simulink model "nms_sim_2D_cost"  (R2024b)
settings: Solver=ode15s  StartTime=0.0  StopTime=t_sim  MaxStep=dt_max  EnableMultiTasking=on
values from neighbouring files (symbols this model uses):
  a_BFSH = param_ctrl(35)*1    [setCtrlPar_optim_CPGreflex2001_2D.m]
  a_GAS = param_ctrl(37)*1    [setCtrlPar_optim_CPGreflex2001_2D.m]
  a_GLU = param_ctrl(31)*1    [setCtrlPar_optim_CPGreflex2001_2D.m]
  a_HAM = param_ctrl(33)*1    [setCtrlPar_optim_CPGreflex2001_2D.m]
  a_HFL = param_ctrl(32)*1    [setCtrlPar_optim_CPGreflex2001_2D.m]
  a_RF = param_ctrl(34)*1    [setCtrlPar_optim_CPGreflex2001_2D.m]
  a_SOL = param_ctrl(38)*1    [setCtrlPar_optim_CPGreflex2001_2D.m]
  a_TA = param_ctrl(39)*1    [setCtrlPar_optim_CPGreflex2001_2D.m]
  a_VAS = param_ctrl(36)*1    [setCtrlPar_optim_CPGreflex2001_2D.m]
  ai = param_ctrl(96)*2.0    [setCtrlPar_optim_CPGreflex2001_2D.m]
  b_BFSH = param_ctrl(52)*.51    [setCtrlPar_optim_CPGreflex2001_2D.m]
  b_BFSHGAS = param_ctrl(55)*.51    [setCtrlPar_optim_CPGreflex2001_2D.m]
  b_BFSHHAM = param_ctrl(54)*.51    [setCtrlPar_optim_CPGreflex2001_2D.m]
  b_BFSHVAS = param_ctrl(53)*.51    [setCtrlPar_optim_CPGreflex2001_2D.m]
  b_GAS = param_ctrl(59)*.51    [setCtrlPar_optim_CPGreflex2001_2D.m]
  b_GASBFSH = param_ctrl(60)*.51    [setCtrlPar_optim_CPGreflex2001_2D.m]
  b_GASSOL = param_ctrl(61)*.51    [setCtrlPar_optim_CPGreflex2001_2D.m]
  b_GLU = param_ctrl(40)*.51    [setCtrlPar_optim_CPGreflex2001_2D.m]
  b_GLUHAM = param_ctrl(42)*.51    [setCtrlPar_optim_CPGreflex2001_2D.m]
  b_GLUHFL = param_ctrl(41)*.51    [setCtrlPar_optim_CPGreflex2001_2D.m]
  b_HAM = param_ctrl(46)*.51    [setCtrlPar_optim_CPGreflex2001_2D.m]
  b_HAMBFSH = param_ctrl(48)*.51    [setCtrlPar_optim_CPGreflex2001_2D.m]
  b_HAMGLU = param_ctrl(47)*.51    [setCtrlPar_optim_CPGreflex2001_2D.m]
  b_HFL = param_ctrl(43)*.51    [setCtrlPar_optim_CPGreflex2001_2D.m]
  b_HFLGLU = param_ctrl(44)*.51    [setCtrlPar_optim_CPGreflex2001_2D.m]
  b_HFLRF = param_ctrl(45)*.51    [setCtrlPar_optim_CPGreflex2001_2D.m]
  b_RF = param_ctrl(49)*.51    [setCtrlPar_optim_CPGreflex2001_2D.m]
  b_RFHFL = param_ctrl(50)*.51    [setCtrlPar_optim_CPGreflex2001_2D.m]
  b_RFVAS = param_ctrl(51)*.51    [setCtrlPar_optim_CPGreflex2001_2D.m]
  b_SOL = param_ctrl(62)*.51    [setCtrlPar_optim_CPGreflex2001_2D.m]
  b_SOLGAS = param_ctrl(64)*.51    [setCtrlPar_optim_CPGreflex2001_2D.m]
  b_SOLTA = param_ctrl(63)*.51    [setCtrlPar_optim_CPGreflex2001_2D.m]
  b_TA = param_ctrl(65)*.51    [setCtrlPar_optim_CPGreflex2001_2D.m]
  b_TASOL = param_ctrl(66)*.51    [setCtrlPar_optim_CPGreflex2001_2D.m]
  b_VAS = param_ctrl(56)*.51    [setCtrlPar_optim_CPGreflex2001_2D.m]
  b_VASBFSH = param_ctrl(57)*.51    [setCtrlPar_optim_CPGreflex2001_2D.m]
  b_VASRF = param_ctrl(58)*.51    [setCtrlPar_optim_CPGreflex2001_2D.m]
  bias = param_ctrl(97)*2.5    [setCtrlPar_optim_CPGreflex2001_2D.m]
  c = 0.05    [nms_MS_2D_scaled.m]
  c_jointstop = 0.3 / (pi/180)    (= 17.1887338539)    [nms_MS_2D_scaled.m]
  D12_F = 0.16    *scaleL_JPhys    [nms_MechInit_2D_scaleSkel.m]
  D12_S = 0.2460	*sub_height    [nms_MechInit_2D_scaleSkel.m]
  D12_T = 0.2450  *sub_height    [nms_MechInit_2D_scaleSkel.m]
  D12y_F = 0.039  *sub_height    [nms_MechInit_2D_scaleSkel.m]
  D12z_HAT = 0.1    [nms_MS_2D_scaled.m]
  D13_F = 0.20    *scaleL_JPhys    [nms_MechInit_2D_scaleSkel.m]
  D1G_F = 0.14    *scaleL_JPhys    [nms_MechInit_2D_scaleSkel.m]
  D1G_HAT = 0.35  *scaleL_JPhys    [nms_MechInit_2D_scaleSkel.m]
  D1G_S = (0.3 - D12y_F/4)	*scaleL_JPhys    [nms_MechInit_2D_scaleSkel.m]
  D1G_T = (0.3 - D12y_F/4)	*scaleL_JPhys    [nms_MechInit_2D_scaleSkel.m]
  D1Gy_F = D12y_F*D1G_F/D12_F    (= 0.07)    [nms_MechInit_2D_scaleSkel.m]
  d_BFSH = param_ctrl(26)*1    [setCtrlPar_optim_CPGreflex2001_2D.m]
  d_GAS = param_ctrl(28)*1    [setCtrlPar_optim_CPGreflex2001_2D.m]
  d_GLU = param_ctrl(22)*1    [setCtrlPar_optim_CPGreflex2001_2D.m]
  d_HAM = param_ctrl(24)*1    [setCtrlPar_optim_CPGreflex2001_2D.m]
  d_HFL = param_ctrl(23)*1    [setCtrlPar_optim_CPGreflex2001_2D.m]
  d_RF = param_ctrl(25)*1    [setCtrlPar_optim_CPGreflex2001_2D.m]
  d_SOL = param_ctrl(29)*1    [setCtrlPar_optim_CPGreflex2001_2D.m]
  d_TA = param_ctrl(30)*1    [setCtrlPar_optim_CPGreflex2001_2D.m]
  d_VAS = param_ctrl(27)*1    [setCtrlPar_optim_CPGreflex2001_2D.m]
  DeltaThRef = 5e-3    (= 0.005)    [nms_MS_2D_scaled.m]
  dloptBFSH = 3.0    (= 3)    [setCtrlPar_optim_CPGreflex2001_2D.m]
  dloptGAS = 3.0    (= 3)    [setCtrlPar_optim_CPGreflex2001_2D.m]
  dloptGLU = 3.0    (= 3)    [setCtrlPar_optim_CPGreflex2001_2D.m]
  dloptHAM = 3.0    (= 3)    [setCtrlPar_optim_CPGreflex2001_2D.m]
  dloptHFL = 3.0    (= 3)    [setCtrlPar_optim_CPGreflex2001_2D.m]
  dloptRF = 3.0    (= 3)    [setCtrlPar_optim_CPGreflex2001_2D.m]
  dloptSOL = 3.0    (= 3)    [setCtrlPar_optim_CPGreflex2001_2D.m]
  dloptTA = 3.0    (= 3)    [setCtrlPar_optim_CPGreflex2001_2D.m]
  dloptVAS = 3.0    (= 3)    [setCtrlPar_optim_CPGreflex2001_2D.m]
  ec_BFSH = param_ctrl(80)*0.15    [setCtrlPar_optim_CPGreflex2001_2D.m]
  ec_GAS = param_ctrl(82)*0.15    [setCtrlPar_optim_CPGreflex2001_2D.m]
  ec_GLU = param_ctrl(76)*0.15    [setCtrlPar_optim_CPGreflex2001_2D.m]
  ec_HAM = param_ctrl(78)*0.15    [setCtrlPar_optim_CPGreflex2001_2D.m]
  ec_HFL = param_ctrl(77)*0.15    [setCtrlPar_optim_CPGreflex2001_2D.m]
  ec_RF = param_ctrl(79)*0.15    [setCtrlPar_optim_CPGreflex2001_2D.m]
  ec_TA = param_ctrl(84)*0.15    [setCtrlPar_optim_CPGreflex2001_2D.m]
  ec_VAS = param_ctrl(81)*0.15    [setCtrlPar_optim_CPGreflex2001_2D.m]
  eref = 0.04    [nms_MS_2D_scaled.m]
  eref_GAS = 0.1    [nms_MS_2D_scaled.m]
  eref_SOL = 0.1    [nms_MS_2D_scaled.m]
  es_BFSH = param_ctrl(89)*0.15    [setCtrlPar_optim_CPGreflex2001_2D.m]
  es_GAS = param_ctrl(91)*0.15    [setCtrlPar_optim_CPGreflex2001_2D.m]
  es_GLU = param_ctrl(85)*0.15    [setCtrlPar_optim_CPGreflex2001_2D.m]
  es_HAM = param_ctrl(87)*0.15    [setCtrlPar_optim_CPGreflex2001_2D.m]
  es_HFL = param_ctrl(86)*0.15    [setCtrlPar_optim_CPGreflex2001_2D.m]
  es_RF = param_ctrl(88)*0.15    [setCtrlPar_optim_CPGreflex2001_2D.m]
  es_TA = param_ctrl(93)*0.15    [setCtrlPar_optim_CPGreflex2001_2D.m]
  es_VAS = param_ctrl(90)*0.15    [setCtrlPar_optim_CPGreflex2001_2D.m]
  FmaxBFSH = 350    [nms_MS_2D_scaled.m]
  FmaxGAS = 2000    [nms_MS_2D_scaled.m]
  FmaxGLU = 4000    [nms_MS_2D_scaled.m]
  FmaxHAM = 2000    [nms_MS_2D_scaled.m]
  FmaxHFL = 2000    [nms_MS_2D_scaled.m]
  FmaxRF = 850    [nms_MS_2D_scaled.m]
  FmaxSOL = 4000    [nms_MS_2D_scaled.m]
  FmaxTA = 800    [nms_MS_2D_scaled.m]
  FmaxVAS = 5000    [nms_MS_2D_scaled.m]
  g = 9.81    [nms_MS_2D_scaled.m]
  gamma_4 = param_ctrl(11) * 1.7    [setCtrlPar_optim_CPGreflexsynergy2023_2D.m]
  h_BFSH = param_ctrl(71)*.1    [setCtrlPar_optim_CPGreflex2001_2D.m]
  h_GAS = param_ctrl(73)*.1    [setCtrlPar_optim_CPGreflex2001_2D.m]
  h_GLU = param_ctrl(67)*.1    [setCtrlPar_optim_CPGreflex2001_2D.m]
  h_HAM = param_ctrl(69)*.1    [setCtrlPar_optim_CPGreflex2001_2D.m]
  h_HFL = param_ctrl(68)*.1    [setCtrlPar_optim_CPGreflex2001_2D.m]
  h_RF = param_ctrl(70)*.1    [setCtrlPar_optim_CPGreflex2001_2D.m]
  h_SOL = param_ctrl(74)*.1    [setCtrlPar_optim_CPGreflex2001_2D.m]
  h_TA = param_ctrl(75)*.1    [setCtrlPar_optim_CPGreflex2001_2D.m]
  h_VAS = param_ctrl(72)*.1    [setCtrlPar_optim_CPGreflex2001_2D.m]
  HLCtrlPar = [theta_tgt l_clr alpha_tgt alpha_cd alpha_cv]    [setCtrlPar_optim_reflex2015_2D.m]
  In_F = 0.005    *scaleM*scaleL_JPhys^2    [nms_MechInit_2D_scaleSkel.m]
  In_HAT = 2.5    *scaleM*scaleL_JPhys^2    [nms_MechInit_2D_scaleSkel.m]
  In_S = 0.05     *scaleM*scaleL_JPhys^2    [nms_MechInit_2D_scaleSkel.m]
  In_T = 0.15     *scaleM*scaleL_JPhys^2    [nms_MechInit_2D_scaleSkel.m]
  init_exc = 0.01    [setInitPar_optim_2D.m]
  init_fm = 0.01    [setInitPar_optim_2D.m]
  init_lce = 1    [setInitPar_optim_2D.m]
  init_LCPG = param_ctrl(12) * 0.01    [setCtrlPar_optim_CPGreflexsynergy2023_2D.m]
  init_LStance = 1    [setInitPar_optim_2D.m]
  init_N1 = osc_signal1(phi_off_osc_ind)    [setCtrlPar_optim_CPGreflex2001_2D.m]
  ... (+441 more)
undefined symbols (not defined in the file or in its folder): cost_act_exponent, cost_v_tgt, flag_controller, Newton, nStep_obj, nStep_startKin, Raphson, sgn, SSW_kin, terrain_slope_angle, v_plateS1, X, Y, Z
libraries: nesl_utility x94, sm_lib x90, simulink x28, simulink_extras x12
(part 11 of 20)

== system nms_sim_2D_cost/Muscle Actuation/L BFSH ==
  note: BFSH Muscle-Tendon Dynamics
  note: Excitation Contraction Coupling
  A : Inport
  lmtc [m] : Inport  Port=2
  1 : Product  Inputs=**  InputSameDT=on  SaturateOnIntegerOverflow=on  OutDataTypeStr=Inherit: Same as first input
  1/lslack : Gain  Gain=1/lslackBFSH  SaturateOnIntegerOverflow=on  OutDataTypeStr=Inherit: Same as input  ParamDataTypeStr=Inherit: Same as input
  BE force-length relation : Subsystem
  CE force-length relation : Subsystem
  CE inverse force-velocity relation : Subsystem
  Constant : Constant  Value=lslackBFSH
  Fmax : Gain  Gain=FmaxBFSH  SaturateOnIntegerOverflow=on  OutDataTypeStr=Inherit: Same as input  ParamDataTypeStr=Inherit: Same as input
  Fmax1 : Gain  Gain=FmaxBFSH  SaturateOnIntegerOverflow=on  OutDataTypeStr=Inherit: Same as input  ParamDataTypeStr=Inherit: Same as input
  "Fpe = F^*pe * fv " : Product  InputSameDT=on  SaturateOnIntegerOverflow=on  OutDataTypeStr=Inherit: Same as first input
  Fv = Fse / (A*Fce) : Product  Inputs=*/  InputSameDT=on  SaturateOnIntegerOverflow=on  OutDataTypeStr=Inherit: Same as first input
  Integrator : Integrator  InitialConditionSource=external  LowerSaturationLimit=0.05
  PE force-length relation : Subsystem
  SE force-length relation : Subsystem
  Sum : Sum  Inputs=|+-  InputSameDT=on  SaturateOnIntegerOverflow=on  OutDataTypeStr=Inherit: Same as first input
  Sum1 : Sum  Inputs=|+-  InputSameDT=on  SaturateOnIntegerOverflow=on  OutDataTypeStr=Inherit: Same as first input
  Sum2 : Sum  Inputs=|-+  InputSameDT=on  SaturateOnIntegerOverflow=on  OutDataTypeStr=Inherit: Same as first input
  Sum3 : Sum  InputSameDT=on  SaturateOnIntegerOverflow=on  OutDataTypeStr=Inherit: Same as first input
  Sum4 : Sum  InputSameDT=on  SaturateOnIntegerOverflow=on  OutDataTypeStr=Inherit: Same as first input
  lce/lopt : Gain  Gain=1/loptBFSH  SaturateOnIntegerOverflow=on  OutDataTypeStr=Inherit: Same as input  ParamDataTypeStr=Inherit: Same as input
  vmax*lopt : Gain  Gain=vmaxBFSH*loptBFSH  SaturateOnIntegerOverflow=on  OutDataTypeStr=Inherit: Same as input  ParamDataTypeStr=Inherit: Same as input
  Fmtc : Outport  InitialOutput=0  VectorParamsAs1DForOutWhenUnconnected=off
  Lce : Outport  Port=2  InitialOutput=0  VectorParamsAs1DForOutWhenUnconnected=off
  Vce : Outport  Port=3  InitialOutput=0  VectorParamsAs1DForOutWhenUnconnected=off
  Fce : Outport  Port=4  InitialOutput=0  VectorParamsAs1DForOutWhenUnconnected=off
  lse [m] : Outport  Port=5  InitialOutput=0  VectorParamsAs1DForOutWhenUnconnected=off
  wires:
  Integrator/1 -> Sum/2, lce/lopt/1, Lce/1  "lce"
  lce/lopt/1 -> CE force-length relation/1(lce [lopt]), PE force-length relation/1(lce [lopt]), BE force-length relation/1(lce [lopt])
  Fv = Fse / (A*Fce)/1 -> "Fpe = F^*pe * fv "/1, CE inverse force-velocity relation/1(Fv[Fmax])  "fv"
  vmax*lopt/1 -> Integrator/1, Vce/1  "vce"
  lmtc [m]/1 -> Sum2/2, Sum/1  "lmtc"
  Fmax/1 -> Fmtc/1  "Fmtc"
  1/lslack/1 -> SE force-length relation/1(lse [lslack])
  SE force-length relation/1(fse [Fmax]) -> Fmax/1, Sum4/1
  Sum2/1 -> Integrator/2
  Constant/1 -> Sum2/1
  CE force-length relation/1(fce [Fmax]) -> 1/1
  PE force-length relation/1(fpe [Fmax]) -> "Fpe = F^*pe * fv "/2, Sum3/1
  1/1 -> Sum3/2
  BE force-length relation/1(fbe [Fmax]) -> Sum4/2
  Sum3/1 -> Fv = Fse / (A*Fce)/2
  CE inverse force-velocity relation/1(v[vmax]) -> vmax*lopt/1
  A/1 -> 1/2
  Sum4/1 -> Sum1/1, Fv = Fse / (A*Fce)/1  "Fse+Fbe"
  "Fpe = F^*pe * fv "/1 -> Sum1/2
  Sum1/1 -> Fmax1/1  "Fse+Fbe-Fpe"
  Fmax1/1 -> Fce/1
  Sum/1 -> lse [m]/1, 1/lslack/1  "lse"

== system nms_sim_2D_cost/Muscle Actuation/L BFSH Link ==
  note: BFSH Attachment
  phi23 [rad] : Inport
  Constant : Constant  Value=lslackBFSH+loptBFSH
  Constant1 : Constant  Value=rBFSH
  Constant2 : Constant  Value=phirefBFSH
  Gain4 : Gain  Gain=rhoBFSH
  Product : Product  RndMeth=Zero
  Sum2 : Sum  Inputs=|+-
  Sum5 : Sum  Inputs=|++
  lmtu [m] : Outport  VectorParamsAs1DForOutWhenUnconnected=off
  lever [m] : Outport  Port=2  VectorParamsAs1DForOutWhenUnconnected=off
  wires:
  Constant/1 -> Sum5/1
  Sum5/1 -> lmtu [m]/1
  Gain4/1 -> Sum5/2
  Product/1 -> Gain4/1
  phi23 [rad]/1 -> Sum2/1
  Constant2/1 -> Sum2/2
  Sum2/1 -> Product/1
  Constant1/1 -> Product/2, lever [m]/1

== system nms_sim_2D_cost/Muscle Actuation/L GAS ==
  note: SOLEUS Muscle-Tendon Dynamics
  note: Excitation Contraction Coupling
  A : Inport
  lmtc [m] : Inport  Port=2
  eref : Inport  Port=3
  1 : Product  Inputs=**  InputSameDT=on  SaturateOnIntegerOverflow=on  OutDataTypeStr=Inherit: Same as first input
  1/lslack : Gain  Gain=1/lslackGAS  SaturateOnIntegerOverflow=on  OutDataTypeStr=Inherit: Same as input  ParamDataTypeStr=Inherit: Same as input
  BE force-length relation : Subsystem
  CE force-length relation : Subsystem
  CE inverse force-velocity relation : Subsystem
  Constant : Constant  Value=lslackGAS
  Fmax : Gain  Gain=FmaxGAS  SaturateOnIntegerOverflow=on  OutDataTypeStr=Inherit: Same as input  ParamDataTypeStr=Inherit: Same as input
  Fmax1 : Gain  Gain=FmaxGAS  SaturateOnIntegerOverflow=on  OutDataTypeStr=Inherit: Same as input  ParamDataTypeStr=Inherit: Same as input
  "Fpe = F^*pe * fv " : Product  InputSameDT=on  SaturateOnIntegerOverflow=on  OutDataTypeStr=Inherit: Same as first input
  Fv = Fse / (A*Fce) : Product  Inputs=*/  InputSameDT=on  SaturateOnIntegerOverflow=on  OutDataTypeStr=Inherit: Same as first input
  Integrator : Integrator  InitialConditionSource=external  LowerSaturationLimit=0.05
  PE force-length relation : Subsystem
  SE force-length relation : Subsystem
  Sum : Sum  Inputs=|+-  InputSameDT=on  SaturateOnIntegerOverflow=on  OutDataTypeStr=Inherit: Same as first input
  Sum1 : Sum  Inputs=|+-  InputSameDT=on  SaturateOnIntegerOverflow=on  OutDataTypeStr=Inherit: Same as first input
  Sum2 : Sum  Inputs=|-+  InputSameDT=on  SaturateOnIntegerOverflow=on  OutDataTypeStr=Inherit: Same as first input
  Sum3 : Sum  InputSameDT=on  SaturateOnIntegerOverflow=on  OutDataTypeStr=Inherit: Same as first input
  Sum4 : Sum  InputSameDT=on  SaturateOnIntegerOverflow=on  OutDataTypeStr=Inherit: Same as first input
  lce/lopt : Gain  Gain=1/loptGAS  SaturateOnIntegerOverflow=on  OutDataTypeStr=Inherit: Same as input  ParamDataTypeStr=Inherit: Same as input
  vmax*lopt : Gain  Gain=vmaxGAS*loptGAS  SaturateOnIntegerOverflow=on  OutDataTypeStr=Inherit: Same as input  ParamDataTypeStr=Inherit: Same as input
  Fmtc : Outport  InitialOutput=0  VectorParamsAs1DForOutWhenUnconnected=off
  Lce : Outport  Port=2  InitialOutput=0  VectorParamsAs1DForOutWhenUnconnected=off
  Vce : Outport  Port=3  InitialOutput=0  VectorParamsAs1DForOutWhenUnconnected=off
  Fce : Outport  Port=4  InitialOutput=0  VectorParamsAs1DForOutWhenUnconnected=off
  lse [m] : Outport  Port=5  InitialOutput=0  VectorParamsAs1DForOutWhenUnconnected=off
  wires:
  Integrator/1 -> Sum/2, lce/lopt/1, Lce/1  "lce"
  lce/lopt/1 -> CE force-length relation/1(lce [lopt]), PE force-length relation/1(lce [lopt]), BE force-length relation/1(lce [lopt])
  Fv = Fse / (A*Fce)/1 -> "Fpe = F^*pe * fv "/1, CE inverse force-velocity relation/1(Fv[Fmax])  "fv"
  vmax*lopt/1 -> Integrator/1, Vce/1  "vce"
  lmtc [m]/1 -> Sum2/2, Sum/1  "lmtc"
  Fmax/1 -> Fmtc/1  "Fmtc"
  1/lslack/1 -> SE force-length relation/1(lse [lslack])
  SE force-length relation/1(fse [Fmax]) -> Fmax/1, Sum4/1
  Sum2/1 -> Integrator/2
  Constant/1 -> Sum2/1
  CE force-length relation/1(fce [Fmax]) -> 1/1
  PE force-length relation/1(fpe [Fmax]) -> "Fpe = F^*pe * fv "/2, Sum3/1
  1/1 -> Sum3/2
  BE force-length relation/1(fbe [Fmax]) -> Sum4/2
  Sum3/1 -> Fv = Fse / (A*Fce)/2
  CE inverse force-velocity relation/1(v[vmax]) -> vmax*lopt/1
  A/1 -> 1/2
  Sum4/1 -> Sum1/1, Fv = Fse / (A*Fce)/1  "Fse+Fbe"
  "Fpe = F^*pe * fv "/1 -> Sum1/2
  Sum1/1 -> Fmax1/1  "Fse+Fbe-Fpe"
  Fmax1/1 -> Fce/1
  Sum/1 -> lse [m]/1, 1/lslack/1  "lse"
  eref/1 -> SE force-length relation/2(eref)

== system nms_sim_2D_cost/Muscle Actuation/L GAS Link ==
  note: GAS Attachment
  phi23 [rad] : Inport
  phi12 [rad] : Inport  Port=2
  Constant1 : Constant  Value=phimaxGASk
  Constant2 : Constant  Value=phirefGASk
  Constant3 : Constant  Value=phimaxGASa
  Constant4 : Constant  Value=lslackGAS+loptGAS
  Constant5 : Constant  Value=phirefGASa
  Demux : Demux  Outputs=2
  Demux1 : Demux  Outputs=2
  Gain1 : Gain  Gain=rGASkmax
  Gain2 : Gain  Gain=rGASamax
  Gain3 : Gain  Gain=phiScaleGASa
  Gain5 : Gain  Gain=phiScaleGASk
  Gain6 : Gain  Gain=phiScaleGASk
  Gain7 : Gain  Gain=rhoGASk/phiScaleGASk
  Gain8 : Gain  Gain=phiScaleGASa
  Gain9 : Gain  Gain=rhoGASa/phiScaleGASa
  Mux : Mux  Inputs=2
  Mux1 : Mux  Inputs=2
  Sum1 : Sum  Inputs=-+
  Sum2 : Sum  Inputs=|+-
  Sum3 : Sum  Inputs=-+|
  Sum4 : Sum  Inputs=-+
  Sum5 : Sum  Inputs=++-
  Sum6 : Sum  Inputs=|+-
  Sum7 : Sum  Inputs=-+|
  length change term : Trigonometry
  length change term1 : Trigonometry
  offset correction term : Trigonometry
  offset correction term1 : Trigonometry
  variable lever term : Trigonometry  Operator=cos
  variable lever term1 : Trigonometry  Operator=cos
  lmtu [m] : Outport  VectorParamsAs1DForOutWhenUnconnected=off
  lever23 [m] : Outport  Port=2  VectorParamsAs1DForOutWhenUnconnected=off
  lever12 [m] : Outport  Port=3  VectorParamsAs1DForOutWhenUnconnected=off
  wires:
  Sum5/1 -> lmtu [m]/1
  Demux1/2 -> lever12 [m]/1
  Constant4/1 -> Sum5/2
  Demux1/1 -> Gain9/1
  Gain9/1 -> Sum5/3
  Demux/2 -> lever23 [m]/1
  Demux/1 -> Gain7/1
  Gain7/1 -> Sum5/1
  phi23 [rad]/1 -> Sum3/2
  Sum3/1 -> Gain5/1
  Constant1/1 -> Sum3/1, Sum2/2
  Sum2/1 -> Gain6/1
  Constant2/1 -> Sum2/1
  length change term/1 -> Sum1/2
  offset correction term/1 -> Sum1/1
  Sum1/1 -> Mux/1
  variable lever term/1 -> Mux/2
  Mux/1 -> Gain1/1
  Gain1/1 -> Demux/1
  Gain5/1 -> variable lever term/1, length change term/1
  Gain6/1 -> offset correction term/1
  phi12 [rad]/1 -> Sum7/2
  Sum7/1 -> Gain3/1
  Constant3/1 -> Sum7/1, Sum6/2
  Sum6/1 -> Gain8/1
  Constant5/1 -> Sum6/1
  length change term1/1 -> Sum4/2
  offset correction term1/1 -> Sum4/1
  Sum4/1 -> Mux1/1
  variable lever term1/1 -> Mux1/2
  Mux1/1 -> Gain2/1
  Gain2/1 -> Demux1/1
  Gain3/1 -> variable lever term1/1, length change term1/1
  Gain8/1 -> offset correction term1/1

== system nms_sim_2D_cost/Muscle Actuation/L Hip Joint Limits ==
  note: Hip Joint Limits
  phi [rad] : Inport
  dphi [rad/s] : Inport  Port=2
  Gain1 : Gain  Gain=c_jointstop
  Gain2 : Gain  Gain=-1
  Gain3 : Gain  Gain=c_jointstop
  Gain4 : Gain  Gain=1/w_max_jointstop
  Limit Ankle Range : simulink/Logic and Bit Operations/Interval Test  Commented=on  IntervalClosedRight=on  uplimit=phi12_UpLimit + 40*pi/180  IntervalClosedLeft=on  lowlimit=phi12_LowLimit - 40*pi/180  OutDataTypeStr=boolean
  Logical Operator3 : Logic  Commented=on  Operator=NOT  AllPortsSameDT=off  OutDataTypeStr=boolean
  Mux1 : Mux  Inputs=2
  Mux3 : Mux  Inputs=2
  Overextension Torque : Fcn  Expr="- u(1)  *  (1-u(2)) * (u(2)<1) * (u(1)>0)"
  Overflexion Torque : Fcn  Expr="- u(1)  *  (1-u(2)) * (u(2)<1) * (u(1)<0)"
  Stop Simulation1 : Stop  Commented=on
  Sum : Sum  Inputs=|+-
  Sum1 : Sum  Inputs=|+-
  Sum2 : Sum
  overextension angle : Constant  Value=phi34_UpLimit
  overflexion angle : Constant  Value=phi34_LowLimit
  M_stop [Nm] : Outport  VectorParamsAs1DForOutWhenUnconnected=off
  wires:
  Mux3/1 -> Overextension Torque/1
  Gain3/1 -> Mux3/1
  dphi [rad/s]/1 -> Gain4/1
  overextension angle/1 -> Sum/2
  phi [rad]/1 -> Sum/1, Sum1/1, Limit Ankle Range/1
  Sum/1 -> Gain3/1
  Gain4/1 -> Gain2/1, Mux1/2
  Gain1/1 -> Mux1/1
  Sum1/1 -> Gain1/1
  overflexion angle/1 -> Sum1/2
  Mux1/1 -> Overflexion Torque/1
  Sum2/1 -> M_stop [Nm]/1
  Gain2/1 -> Mux3/2
  Overflexion Torque/1 -> Sum2/2
  Overextension Torque/1 -> Sum2/1
  Limit Ankle Range/1 -> Logical Operator3/1
  Logical Operator3/1 -> Stop Simulation1/1

== system nms_sim_2D_cost/Muscle Actuation/L Knee Joint Limits ==
  note: Knee Joint Limits
  phi [rad] : Inport
  dphi [rad/s] : Inport  Port=2
  Gain1 : Gain  Gain=c_jointstop
  Gain2 : Gain  Gain=-1
  Gain3 : Gain  Gain=c_jointstop
  Gain4 : Gain  Gain=1/w_max_jointstop
  Limit Ankle Range : simulink/Logic and Bit Operations/Interval Test  Commented=on  IntervalClosedRight=on  uplimit=phi12_UpLimit + 40*pi/180  IntervalClosedLeft=on  lowlimit=phi12_LowLimit - 40*pi/180  OutDataTypeStr=boolean
  Logical Operator3 : Logic  Commented=on  Operator=NOT  AllPortsSameDT=off  OutDataTypeStr=boolean
  Mux1 : Mux  Inputs=2
  Mux3 : Mux  Inputs=2
  Overextension Torque : Fcn  Expr="- u(1)  *  (1-u(2)) * (u(2)<1) * (u(1)>0)"
  Overflexion Torque : Fcn  Expr="- u(1)  *  (1-u(2)) * (u(2)<1) * (u(1)<0)"
  Stop Simulation1 : Stop  Commented=on
  Sum : Sum  Inputs=|+-
  Sum1 : Sum  Inputs=|+-
  Sum2 : Sum
  overextension angle : Constant  Value=phi23_UpLimit
  overflexion angle : Constant  Value=phi23_LowLimit
  M_stop [Nm] : Outport  VectorParamsAs1DForOutWhenUnconnected=off
  wires:
  Mux3/1 -> Overextension Torque/1
  Gain3/1 -> Mux3/1
  dphi [rad/s]/1 -> Gain4/1
  overextension angle/1 -> Sum/2
  phi [rad]/1 -> Sum/1, Sum1/1, Limit Ankle Range/1
  Sum/1 -> Gain3/1
  Gain4/1 -> Gain2/1, Mux1/2
  Gain1/1 -> Mux1/1
  Sum1/1 -> Gain1/1
  overflexion angle/1 -> Sum1/2
  Mux1/1 -> Overflexion Torque/1
  Sum2/1 -> M_stop [Nm]/1
  Gain2/1 -> Mux3/2
  Overflexion Torque/1 -> Sum2/2
  Overextension Torque/1 -> Sum2/1
  Limit Ankle Range/1 -> Logical Operator3/1
  Logical Operator3/1 -> Stop Simulation1/1

== system nms_sim_2D_cost/Muscle Actuation/L SOL ==
  note: SOLEUS Muscle-Tendon Dynamics
  note: Excitation Contraction Coupling
  A : Inport
  lmtc [m] : Inport  Port=2
  eref : Inport  Port=3
  1 : Product  Inputs=**  InputSameDT=on  SaturateOnIntegerOverflow=on  OutDataTypeStr=Inherit: Same as first input
  1/lslack : Gain  Gain=1/lslackSOL  SaturateOnIntegerOverflow=on  OutDataTypeStr=Inherit: Same as input  ParamDataTypeStr=Inherit: Same as input
  BE force-length relation : Subsystem
  CE force-length relation : Subsystem
  CE inverse force-velocity relation : Subsystem
  Constant : Constant  Value=lslackSOL
  Fmax : Gain  Gain=FmaxSOL  SaturateOnIntegerOverflow=on  OutDataTypeStr=Inherit: Same as input  ParamDataTypeStr=Inherit: Same as input
  Fmax1 : Gain  Gain=FmaxSOL  SaturateOnIntegerOverflow=on  OutDataTypeStr=Inherit: Same as input  ParamDataTypeStr=Inherit: Same as input
  "Fpe = F^*pe * fv " : Product  InputSameDT=on  SaturateOnIntegerOverflow=on  OutDataTypeStr=Inherit: Same as first input
  Fv = Fse / (A*Fce) : Product  Inputs=*/  InputSameDT=on  SaturateOnIntegerOverflow=on  OutDataTypeStr=Inherit: Same as first input
  Integrator : Integrator  InitialConditionSource=external  LowerSaturationLimit=0.05
  PE force-length relation : Subsystem
  SE force-length relation : Subsystem
  Sum : Sum  Inputs=|+-  InputSameDT=on  SaturateOnIntegerOverflow=on  OutDataTypeStr=Inherit: Same as first input
  Sum1 : Sum  Inputs=|+-  InputSameDT=on  SaturateOnIntegerOverflow=on  OutDataTypeStr=Inherit: Same as first input
  Sum2 : Sum  Inputs=|-+  InputSameDT=on  SaturateOnIntegerOverflow=on  OutDataTypeStr=Inherit: Same as first input
  Sum3 : Sum  InputSameDT=on  SaturateOnIntegerOverflow=on  OutDataTypeStr=Inherit: Same as first input
  Sum4 : Sum  InputSameDT=on  SaturateOnIntegerOverflow=on  OutDataTypeStr=Inherit: Same as first input
  lce/lopt : Gain  Gain=1/loptSOL  SaturateOnIntegerOverflow=on  OutDataTypeStr=Inherit: Same as input  ParamDataTypeStr=Inherit: Same as input
  vmax*lopt : Gain  Gain=vmaxSOL*loptSOL  SaturateOnIntegerOverflow=on  OutDataTypeStr=Inherit: Same as input  ParamDataTypeStr=Inherit: Same as input
  Fmtc : Outport  InitialOutput=0  VectorParamsAs1DForOutWhenUnconnected=off
  Lce : Outport  Port=2  InitialOutput=0  VectorParamsAs1DForOutWhenUnconnected=off
  Vce : Outport  Port=3  InitialOutput=0  VectorParamsAs1DForOutWhenUnconnected=off
  Fce : Outport  Port=4  InitialOutput=0  VectorParamsAs1DForOutWhenUnconnected=off
  lse [m] : Outport  Port=5  InitialOutput=0  VectorParamsAs1DForOutWhenUnconnected=off
  wires:
  Integrator/1 -> Sum/2, lce/lopt/1, Lce/1  "lce"
  lce/lopt/1 -> CE force-length relation/1(lce [lopt]), PE force-length relation/1(lce [lopt]), BE force-length relation/1(lce [lopt])
  Fv = Fse / (A*Fce)/1 -> "Fpe = F^*pe * fv "/1, CE inverse force-velocity relation/1(Fv[Fmax])  "fv"
  vmax*lopt/1 -> Integrator/1, Vce/1  "vce"
  lmtc [m]/1 -> Sum2/2, Sum/1  "lmtc"
  Fmax/1 -> Fmtc/1  "Fmtc"
  1/lslack/1 -> SE force-length relation/1(lse [lslack])
  SE force-length relation/1(fse [Fmax]) -> Fmax/1, Sum4/1
  Sum2/1 -> Integrator/2
  Constant/1 -> Sum2/1
  CE force-length relation/1(fce [Fmax]) -> 1/1
  PE force-length relation/1(fpe [Fmax]) -> "Fpe = F^*pe * fv "/2, Sum3/1
  1/1 -> Sum3/2
  BE force-length relation/1(fbe [Fmax]) -> Sum4/2
  Sum3/1 -> Fv = Fse / (A*Fce)/2
  CE inverse force-velocity relation/1(v[vmax]) -> vmax*lopt/1
  A/1 -> 1/2
  Sum4/1 -> Sum1/1, Fv = Fse / (A*Fce)/1  "Fse+Fbe"
  "Fpe = F^*pe * fv "/1 -> Sum1/2
  Sum1/1 -> Fmax1/1  "Fse+Fbe-Fpe"
  Fmax1/1 -> Fce/1
  Sum/1 -> lse [m]/1, 1/lslack/1  "lse"
  eref/1 -> SE force-length relation/2(eref)

== system nms_sim_2D_cost/Muscle Actuation/L SOL Link ==
  note: Soleus Attachment
  phi12 [rad] : Inport
  Constant : Constant  Value=lslackSOL+loptSOL
  Constant3 : Constant  Value=phimaxSOL
  Constant5 : Constant  Value=phirefSOL
  Demux1 : Demux  Outputs=2
  Gain2 : Gain  Gain=rSOLmax
  Gain3 : Gain  Gain=phiScaleSOL
  Gain8 : Gain  Gain=phiScaleSOL
  Gain9 : Gain  Gain=rhoSOL/phiScaleSOL
  Mux1 : Mux  Inputs=2
  Sum4 : Sum  Inputs=-+
  Sum5 : Sum  Inputs=|+-
  Sum6 : Sum  Inputs=|+-
  Sum7 : Sum  Inputs=-+|
  length change term1 : Trigonometry
  offset correction term1 : Trigonometry
  variable lever term1 : Trigonometry  Operator=cos
  lmtc [m] : Outport  VectorParamsAs1DForOutWhenUnconnected=off
  lever [m] : Outport  Port=2  VectorParamsAs1DForOutWhenUnconnected=off
  wires:
  Constant/1 -> Sum5/1
  Sum5/1 -> lmtc [m]/1
  Gain9/1 -> Sum5/2
  Demux1/1 -> Gain9/1
  Demux1/2 -> lever [m]/1
  phi12 [rad]/1 -> Sum7/2
  Sum7/1 -> Gain3/1
  Constant3/1 -> Sum7/1, Sum6/2
  Sum6/1 -> Gain8/1
  Constant5/1 -> Sum6/1
  length change term1/1 -> Sum4/2
  offset correction term1/1 -> Sum4/1
  Sum4/1 -> Mux1/1
  variable lever term1/1 -> Mux1/2
  Mux1/1 -> Gain2/1
  Gain2/1 -> Demux1/1
  Gain3/1 -> variable lever term1/1, length change term1/1
  Gain8/1 -> offset correction term1/1

== system nms_sim_2D_cost/Muscle Actuation/L TA ==
  note: Excitation Contraction Coupling
  note: SOLEUS Muscle-Tendon Dynamics
  A : Inport
  lmtc [m] : Inport  Port=2
  1 : Product  Inputs=**  InputSameDT=on  SaturateOnIntegerOverflow=on  OutDataTypeStr=Inherit: Same as first input
  1/lslack : Gain  Gain=1/lslackTA  SaturateOnIntegerOverflow=on  OutDataTypeStr=Inherit: Same as input  ParamDataTypeStr=Inherit: Same as input
  BE force-length relation : Subsystem
  CE force-length relation : Subsystem
  CE inverse force-velocity relation : Subsystem
  Constant : Constant  Value=lslackTA
  Fmax : Gain  Gain=FmaxTA  SaturateOnIntegerOverflow=on  OutDataTypeStr=Inherit: Same as input  ParamDataTypeStr=Inherit: Same as input
  Fmax1 : Gain  Gain=FmaxTA  SaturateOnIntegerOverflow=on  OutDataTypeStr=Inherit: Same as input  ParamDataTypeStr=Inherit: Same as input
  "Fpe = F^*pe * fv " : Product  InputSameDT=on  SaturateOnIntegerOverflow=on  OutDataTypeStr=Inherit: Same as first input
  Fv = Fse / (A*Fce) : Product  Inputs=*/  InputSameDT=on  SaturateOnIntegerOverflow=on  OutDataTypeStr=Inherit: Same as first input
  Integrator : Integrator  InitialConditionSource=external  LowerSaturationLimit=0.05
  PE force-length relation : Subsystem
  SE force-length relation : Subsystem
  Sum : Sum  Inputs=|+-  InputSameDT=on  SaturateOnIntegerOverflow=on  OutDataTypeStr=Inherit: Same as first input
  Sum1 : Sum  Inputs=|+-  InputSameDT=on  SaturateOnIntegerOverflow=on  OutDataTypeStr=Inherit: Same as first input
  Sum2 : Sum  Inputs=|-+  InputSameDT=on  SaturateOnIntegerOverflow=on  OutDataTypeStr=Inherit: Same as first input
  Sum3 : Sum  InputSameDT=on  SaturateOnIntegerOverflow=on  OutDataTypeStr=Inherit: Same as first input
  Sum4 : Sum  InputSameDT=on  SaturateOnIntegerOverflow=on  OutDataTypeStr=Inherit: Same as first input
  lce/lopt : Gain  Gain=1/loptTA  SaturateOnIntegerOverflow=on  OutDataTypeStr=Inherit: Same as input  ParamDataTypeStr=Inherit: Same as input
  vmax*lopt : Gain  Gain=vmaxTA*loptTA  SaturateOnIntegerOverflow=on  OutDataTypeStr=Inherit: Same as input  ParamDataTypeStr=Inherit: Same as input
  Fmtc : Outport  InitialOutput=0  VectorParamsAs1DForOutWhenUnconnected=off
  Lce : Outport  Port=2  InitialOutput=0  VectorParamsAs1DForOutWhenUnconnected=off
  Vce : Outport  Port=3  InitialOutput=0  VectorParamsAs1DForOutWhenUnconnected=off
  Fce : Outport  Port=4  InitialOutput=0  VectorParamsAs1DForOutWhenUnconnected=off
  lse [m] : Outport  Port=5  InitialOutput=0  VectorParamsAs1DForOutWhenUnconnected=off
  wires:
  CE inverse force-velocity relation/1(v[vmax]) -> vmax*lopt/1
  Sum3/1 -> Fv = Fse / (A*Fce)/2
  BE force-length relation/1(fbe [Fmax]) -> Sum4/2
  1/1 -> Sum3/2
  PE force-length relation/1(fpe [Fmax]) -> "Fpe = F^*pe * fv "/2, Sum3/1
  CE force-length relation/1(fce [Fmax]) -> 1/1
  Constant/1 -> Sum2/1
  Sum2/1 -> Integrator/2
  SE force-length relation/1(fse [Fmax]) -> Sum4/1, Fmax/1
  1/lslack/1 -> SE force-length relation/1(lse [lslack])
  Fmax/1 -> Fmtc/1  "Fmtc"
  lmtc [m]/1 -> Sum/1, Sum2/2  "lmtc"
  vmax*lopt/1 -> Integrator/1, Vce/1  "vce"
  Fv = Fse / (A*Fce)/1 -> "Fpe = F^*pe * fv "/1, CE inverse force-velocity relation/1(Fv[Fmax])  "fv"
  lce/lopt/1 -> PE force-length relation/1(lce [lopt]), BE force-length relation/1(lce [lopt]), CE force-length relation/1(lce [lopt])
  Integrator/1 -> lce/lopt/1, Sum/2, Lce/1  "lce"
  A/1 -> 1/2
  Sum4/1 -> Sum1/1, Fv = Fse / (A*Fce)/1  "Fse+Fbe"
  "Fpe = F^*pe * fv "/1 -> Sum1/2
  Sum1/1 -> Fmax1/1  "Fse+Fbe-Fpe"
  Fmax1/1 -> Fce/1
  Sum/1 -> lse [m]/1, 1/lslack/1  "lse"

== system nms_sim_2D_cost/Muscle Actuation/L TA Link ==
  note: Muscle Length and Moment Arm
  phi12 [rad] : Inport
  Constant : Constant  Value=lslackTA+loptTA
  Constant3 : Constant  Value=phimaxTA
  Constant5 : Constant  Value=phirefTA
  Demux1 : Demux  Outputs=2
  Gain2 : Gain  Gain=rTAmax
  Gain3 : Gain  Gain=phiScaleTA
  Gain8 : Gain  Gain=phiScaleTA
  Gain9 : Gain  Gain=rhoTA/phiScaleTA
  Mux1 : Mux  Inputs=2
  Sum4 : Sum  Inputs=-+
  Sum5 : Sum  Inputs=|++
  Sum6 : Sum  Inputs=|+-
  Sum7 : Sum  Inputs=-+|
  length change term1 : Trigonometry
  offset correction term1 : Trigonometry
  variable lever term1 : Trigonometry  Operator=cos
  lmtc [m] : Outport  VectorParamsAs1DForOutWhenUnconnected=off
  lever [m] : Outport  Port=2  VectorParamsAs1DForOutWhenUnconnected=off
  wires:
  Constant/1 -> Sum5/1
  Sum5/1 -> lmtc [m]/1
  Gain9/1 -> Sum5/2
  Demux1/1 -> Gain9/1
  Demux1/2 -> lever [m]/1
  phi12 [rad]/1 -> Sum7/2
  Sum7/1 -> Gain3/1
  Constant3/1 -> Sum7/1, Sum6/2
  Sum6/1 -> Gain8/1
  Constant5/1 -> Sum6/1
  length change term1/1 -> Sum4/2
  offset correction term1/1 -> Sum4/1
  Sum4/1 -> Mux1/1
  variable lever term1/1 -> Mux1/2
  Mux1/1 -> Gain2/1
  Gain2/1 -> Demux1/1
  Gain3/1 -> variable lever term1/1, length change term1/1
  Gain8/1 -> offset correction term1/1

== system nms_sim_2D_cost/Muscle Actuation/R Ankle Joint Limits ==
  note: Ankle Joint Limits
  phi [rad] : Inport
  dphi [rad/s] : Inport  Port=2
  Gain1 : Gain  Gain=c_jointstop
  Gain2 : Gain  Gain=-1
  Gain3 : Gain  Gain=c_jointstop
  Gain4 : Gain  Gain=1/w_max_jointstop
  Limit Ankle Range : simulink/Logic and Bit Operations/Interval Test  Commented=on  IntervalClosedRight=on  uplimit=phi12_UpLimit + 40*pi/180  IntervalClosedLeft=on  lowlimit=phi12_LowLimit - 40*pi/180  OutDataTypeStr=boolean
  Logical Operator3 : Logic  Commented=on  Operator=NOT  AllPortsSameDT=off  OutDataTypeStr=boolean
  Mux1 : Mux  Inputs=2
  Mux3 : Mux  Inputs=2
  Overextension Torque : Fcn  Expr="- u(1)  *  (1-u(2)) * (u(2)<1) * (u(1)>0)"
  Overflexion Torque : Fcn  Expr="- u(1)  *  (1-u(2)) * (u(2)<1) * (u(1)<0)"
  Stop Simulation1 : Stop  Commented=on
  Sum : Sum  Inputs=|+-
  Sum1 : Sum  Inputs=|+-
  Sum2 : Sum
  overextension angle : Constant  Value=phi12_UpLimit
  overflexion angle : Constant  Value=phi12_LowLimit
  M_stop [Nm] : Outport  VectorParamsAs1DForOutWhenUnconnected=off
  wires:
  Mux3/1 -> Overextension Torque/1
  Gain3/1 -> Mux3/1
  dphi [rad/s]/1 -> Gain4/1
  overextension angle/1 -> Sum/2
  phi [rad]/1 -> Sum/1, Sum1/1, Limit Ankle Range/1
  Sum/1 -> Gain3/1
  Gain4/1 -> Gain2/1, Mux1/2
  Gain1/1 -> Mux1/1
  Sum1/1 -> Gain1/1
  overflexion angle/1 -> Sum1/2
  Mux1/1 -> Overflexion Torque/1
  Sum2/1 -> M_stop [Nm]/1
  Gain2/1 -> Mux3/2
  Overflexion Torque/1 -> Sum2/2
  Overextension Torque/1 -> Sum2/1
  Limit Ankle Range/1 -> Logical Operator3/1
  Logical Operator3/1 -> Stop Simulation1/1

== system nms_sim_2D_cost/Muscle Actuation/R BFSH ==
  note: BFSH Muscle-Tendon Dynamics
  note: Excitation Contraction Coupling
  A : Inport
  lmtc [m] : Inport  Port=2
  1 : Product  Inputs=**  InputSameDT=on  SaturateOnIntegerOverflow=on  OutDataTypeStr=Inherit: Same as first input
  1/lslack : Gain  Gain=1/lslackBFSH  SaturateOnIntegerOverflow=on  OutDataTypeStr=Inherit: Same as input  ParamDataTypeStr=Inherit: Same as input
  BE force-length relation : Subsystem
  CE force-length relation : Subsystem
  CE inverse force-velocity relation : Subsystem
  Constant : Constant  Value=lslackBFSH
  Fmax : Gain  Gain=FmaxBFSH  SaturateOnIntegerOverflow=on  OutDataTypeStr=Inherit: Same as input  ParamDataTypeStr=Inherit: Same as input
  Fmax1 : Gain  Gain=FmaxBFSH  SaturateOnIntegerOverflow=on  OutDataTypeStr=Inherit: Same as input  ParamDataTypeStr=Inherit: Same as input
  "Fpe = F^*pe * fv " : Product  InputSameDT=on  SaturateOnIntegerOverflow=on  OutDataTypeStr=Inherit: Same as first input
  Fv = Fse / (A*Fce) : Product  Inputs=*/  InputSameDT=on  SaturateOnIntegerOverflow=on  OutDataTypeStr=Inherit: Same as first input
  Integrator : Integrator  InitialConditionSource=external  LowerSaturationLimit=0.05
  PE force-length relation : Subsystem
  SE force-length relation : Subsystem
  Sum : Sum  Inputs=|+-  InputSameDT=on  SaturateOnIntegerOverflow=on  OutDataTypeStr=Inherit: Same as first input
  Sum1 : Sum  Inputs=|+-  InputSameDT=on  SaturateOnIntegerOverflow=on  OutDataTypeStr=Inherit: Same as first input
  Sum2 : Sum  Inputs=|-+  InputSameDT=on  SaturateOnIntegerOverflow=on  OutDataTypeStr=Inherit: Same as first input
  Sum3 : Sum  InputSameDT=on  SaturateOnIntegerOverflow=on  OutDataTypeStr=Inherit: Same as first input
  Sum4 : Sum  InputSameDT=on  SaturateOnIntegerOverflow=on  OutDataTypeStr=Inherit: Same as first input
  lce/lopt : Gain  Gain=1/loptBFSH  SaturateOnIntegerOverflow=on  OutDataTypeStr=Inherit: Same as input  ParamDataTypeStr=Inherit: Same as input
  vmax*lopt : Gain  Gain=vmaxBFSH*loptBFSH  SaturateOnIntegerOverflow=on  OutDataTypeStr=Inherit: Same as input  ParamDataTypeStr=Inherit: Same as input
  Fmtc : Outport  InitialOutput=0  VectorParamsAs1DForOutWhenUnconnected=off
  Lce : Outport  Port=2  InitialOutput=0  VectorParamsAs1DForOutWhenUnconnected=off
  Vce : Outport  Port=3  InitialOutput=0  VectorParamsAs1DForOutWhenUnconnected=off
  Fce : Outport  Port=4  InitialOutput=0  VectorParamsAs1DForOutWhenUnconnected=off
  lse [m] : Outport  Port=5  InitialOutput=0  VectorParamsAs1DForOutWhenUnconnected=off
  wires:
  Integrator/1 -> Sum/2, lce/lopt/1, Lce/1  "lce"
  lce/lopt/1 -> CE force-length relation/1(lce [lopt]), PE force-length relation/1(lce [lopt]), BE force-length relation/1(lce [lopt])
  Fv = Fse / (A*Fce)/1 -> "Fpe = F^*pe * fv "/1, CE inverse force-velocity relation/1(Fv[Fmax])  "fv"
  vmax*lopt/1 -> Integrator/1, Vce/1  "vce"
  lmtc [m]/1 -> Sum2/2, Sum/1  "lmtc"
  Fmax/1 -> Fmtc/1  "Fmtc"
  1/lslack/1 -> SE force-length relation/1(lse [lslack])
  SE force-length relation/1(fse [Fmax]) -> Fmax/1, Sum4/1
  Sum2/1 -> Integrator/2
  Constant/1 -> Sum2/1
  CE force-length relation/1(fce [Fmax]) -> 1/1
  PE force-length relation/1(fpe [Fmax]) -> "Fpe = F^*pe * fv "/2, Sum3/1
  1/1 -> Sum3/2
  BE force-length relation/1(fbe [Fmax]) -> Sum4/2
  Sum3/1 -> Fv = Fse / (A*Fce)/2
  CE inverse force-velocity relation/1(v[vmax]) -> vmax*lopt/1
  A/1 -> 1/2
  Sum4/1 -> Sum1/1, Fv = Fse / (A*Fce)/1  "Fse+Fbe"
  "Fpe = F^*pe * fv "/1 -> Sum1/2
  Sum1/1 -> Fmax1/1  "Fse+Fbe-Fpe"
  Fmax1/1 -> Fce/1
  Sum/1 -> lse [m]/1, 1/lslack/1  "lse"

== system nms_sim_2D_cost/Muscle Actuation/R BFSH Link ==
  note: BFSH Attachment
  phi23 [rad] : Inport
  Constant : Constant  Value=lslackBFSH+loptBFSH
  Constant1 : Constant  Value=rBFSH
  Constant2 : Constant  Value=phirefBFSH
  Gain4 : Gain  Gain=rhoBFSH
  Product : Product  RndMeth=Zero
  Sum2 : Sum  Inputs=|+-
  Sum5 : Sum  Inputs=|++
  lmtu [m] : Outport  VectorParamsAs1DForOutWhenUnconnected=off
  lever [m] : Outport  Port=2  VectorParamsAs1DForOutWhenUnconnected=off
  wires:
  Constant/1 -> Sum5/1
  Sum5/1 -> lmtu [m]/1
  Gain4/1 -> Sum5/2
  Product/1 -> Gain4/1
  phi23 [rad]/1 -> Sum2/1
  Constant2/1 -> Sum2/2
  Sum2/1 -> Product/1
  Constant1/1 -> Product/2, lever [m]/1

== system nms_sim_2D_cost/Muscle Actuation/R GAS ==
  note: SOLEUS Muscle-Tendon Dynamics
  note: Excitation Contraction Coupling
  A : Inport
  lmtc [m] : Inport  Port=2
  eref : Inport  Port=3
  1 : Product  Inputs=**  InputSameDT=on  SaturateOnIntegerOverflow=on  OutDataTypeStr=Inherit: Same as first input
  1/lslack : Gain  Gain=1/lslackGAS  SaturateOnIntegerOverflow=on  OutDataTypeStr=Inherit: Same as input  ParamDataTypeStr=Inherit: Same as input
  BE force-length relation : Subsystem
  CE force-length relation : Subsystem
  CE inverse force-velocity relation : Subsystem
  Constant : Constant  Value=lslackGAS
  Fmax : Gain  Gain=FmaxGAS  SaturateOnIntegerOverflow=on  OutDataTypeStr=Inherit: Same as input  ParamDataTypeStr=Inherit: Same as input
  Fmax1 : Gain  Gain=FmaxGAS  SaturateOnIntegerOverflow=on  OutDataTypeStr=Inherit: Same as input  ParamDataTypeStr=Inherit: Same as input
  "Fpe = F^*pe * fv " : Product  InputSameDT=on  SaturateOnIntegerOverflow=on  OutDataTypeStr=Inherit: Same as first input
  Fv = Fse / (A*Fce) : Product  Inputs=*/  InputSameDT=on  SaturateOnIntegerOverflow=on  OutDataTypeStr=Inherit: Same as first input
  Integrator : Integrator  InitialConditionSource=external  LowerSaturationLimit=0.05
  PE force-length relation : Subsystem
  SE force-length relation : Subsystem
  Sum : Sum  Inputs=|+-  InputSameDT=on  SaturateOnIntegerOverflow=on  OutDataTypeStr=Inherit: Same as first input
  Sum1 : Sum  Inputs=|+-  InputSameDT=on  SaturateOnIntegerOverflow=on  OutDataTypeStr=Inherit: Same as first input
  Sum2 : Sum  Inputs=|-+  InputSameDT=on  SaturateOnIntegerOverflow=on  OutDataTypeStr=Inherit: Same as first input
  Sum3 : Sum  InputSameDT=on  SaturateOnIntegerOverflow=on  OutDataTypeStr=Inherit: Same as first input
  Sum4 : Sum  InputSameDT=on  SaturateOnIntegerOverflow=on  OutDataTypeStr=Inherit: Same as first input
  lce/lopt : Gain  Gain=1/loptGAS  SaturateOnIntegerOverflow=on  OutDataTypeStr=Inherit: Same as input  ParamDataTypeStr=Inherit: Same as input
  vmax*lopt : Gain  Gain=vmaxGAS*loptGAS  SaturateOnIntegerOverflow=on  OutDataTypeStr=Inherit: Same as input  ParamDataTypeStr=Inherit: Same as input
  Fmtc : Outport  InitialOutput=0  VectorParamsAs1DForOutWhenUnconnected=off
  Lce : Outport  Port=2  InitialOutput=0  VectorParamsAs1DForOutWhenUnconnected=off
  Vce : Outport  Port=3  InitialOutput=0  VectorParamsAs1DForOutWhenUnconnected=off
  Fce : Outport  Port=4  InitialOutput=0  VectorParamsAs1DForOutWhenUnconnected=off
  lse [m] : Outport  Port=5  InitialOutput=0  VectorParamsAs1DForOutWhenUnconnected=off
  wires:
  Integrator/1 -> Sum/2, lce/lopt/1, Lce/1  "lce"
  lce/lopt/1 -> CE force-length relation/1(lce [lopt]), PE force-length relation/1(lce [lopt]), BE force-length relation/1(lce [lopt])
  Fv = Fse / (A*Fce)/1 -> "Fpe = F^*pe * fv "/1, CE inverse force-velocity relation/1(Fv[Fmax])  "fv"
  vmax*lopt/1 -> Integrator/1, Vce/1  "vce"
  lmtc [m]/1 -> Sum2/2, Sum/1  "lmtc"
  Fmax/1 -> Fmtc/1  "Fmtc"
  1/lslack/1 -> SE force-length relation/1(lse [lslack])
  SE force-length relation/1(fse [Fmax]) -> Fmax/1, Sum4/1
  Sum2/1 -> Integrator/2
  Constant/1 -> Sum2/1
  CE force-length relation/1(fce [Fmax]) -> 1/1
  PE force-length relation/1(fpe [Fmax]) -> "Fpe = F^*pe * fv "/2, Sum3/1
  1/1 -> Sum3/2
  BE force-length relation/1(fbe [Fmax]) -> Sum4/2
  Sum3/1 -> Fv = Fse / (A*Fce)/2
  CE inverse force-velocity relation/1(v[vmax]) -> vmax*lopt/1
  A/1 -> 1/2
  Sum4/1 -> Sum1/1, Fv = Fse / (A*Fce)/1  "Fse+Fbe"
  "Fpe = F^*pe * fv "/1 -> Sum1/2
  Sum1/1 -> Fmax1/1  "Fse+Fbe-Fpe"
  Fmax1/1 -> Fce/1
  Sum/1 -> lse [m]/1, 1/lslack/1  "lse"
  eref/1 -> SE force-length relation/2(eref)

== system nms_sim_2D_cost/Muscle Actuation/R GAS Link ==
  note: GAS Attachment
  phi23 [rad] : Inport
  phi12 [rad] : Inport  Port=2
  Constant1 : Constant  Value=phimaxGASk
  Constant2 : Constant  Value=phirefGASk
  Constant3 : Constant  Value=phimaxGASa
  Constant4 : Constant  Value=lslackGAS+loptGAS
  Constant5 : Constant  Value=phirefGASa
  Demux : Demux  Outputs=2
  Demux1 : Demux  Outputs=2
  Gain1 : Gain  Gain=rGASkmax
  Gain2 : Gain  Gain=rGASamax
  Gain3 : Gain  Gain=phiScaleGASa
  Gain5 : Gain  Gain=phiScaleGASk
  Gain6 : Gain  Gain=phiScaleGASk
  Gain7 : Gain  Gain=rhoGASk/phiScaleGASk
  Gain8 : Gain  Gain=phiScaleGASa
  Gain9 : Gain  Gain=rhoGASa/phiScaleGASa
  Mux : Mux  Inputs=2
  Mux1 : Mux  Inputs=2
  Sum1 : Sum  Inputs=-+
  Sum2 : Sum  Inputs=|+-
  Sum3 : Sum  Inputs=-+|
  Sum4 : Sum  Inputs=-+
  Sum5 : Sum  Inputs=++-
  Sum6 : Sum  Inputs=|+-
  Sum7 : Sum  Inputs=-+|
  length change term : Trigonometry
  length change term1 : Trigonometry
  offset correction term : Trigonometry
  offset correction term1 : Trigonometry
  variable lever term : Trigonometry  Operator=cos
  variable lever term1 : Trigonometry  Operator=cos
  lmtu [m] : Outport  VectorParamsAs1DForOutWhenUnconnected=off
  lever23 [m] : Outport  Port=2  VectorParamsAs1DForOutWhenUnconnected=off
  lever12 [m] : Outport  Port=3  VectorParamsAs1DForOutWhenUnconnected=off
  wires:
  Sum5/1 -> lmtu [m]/1
  Demux1/2 -> lever12 [m]/1
  Constant4/1 -> Sum5/2
  Demux1/1 -> Gain9/1
  Gain9/1 -> Sum5/3
  Demux/2 -> lever23 [m]/1
  Demux/1 -> Gain7/1
  Gain7/1 -> Sum5/1
  phi23 [rad]/1 -> Sum3/2
  Sum3/1 -> Gain5/1
  Constant1/1 -> Sum3/1, Sum2/2
  Sum2/1 -> Gain6/1
  Constant2/1 -> Sum2/1
  length change term/1 -> Sum1/2
  offset correction term/1 -> Sum1/1
  Sum1/1 -> Mux/1
  variable lever term/1 -> Mux/2
  Mux/1 -> Gain1/1
  Gain1/1 -> Demux/1
  Gain5/1 -> variable lever term/1, length change term/1
  Gain6/1 -> offset correction term/1
  phi12 [rad]/1 -> Sum7/2
  Sum7/1 -> Gain3/1
  Constant3/1 -> Sum7/1, Sum6/2
  Sum6/1 -> Gain8/1
  Constant5/1 -> Sum6/1
  length change term1/1 -> Sum4/2
  offset correction term1/1 -> Sum4/1
  Sum4/1 -> Mux1/1
  variable lever term1/1 -> Mux1/2
  Mux1/1 -> Gain2/1
  Gain2/1 -> Demux1/1
  Gain3/1 -> variable lever term1/1, length change term1/1
  Gain8/1 -> offset correction term1/1

== system nms_sim_2D_cost/Muscle Actuation/R GLU Link ==
  note: GLUTEUS Attachment
  phi34 [rad] : Inport
  Constant : Constant  Value=lslackGLU+loptGLU
  Constant1 : Constant  Value=rGLU
  Constant2 : Constant  Value=phirefGLU
  Gain2 : Gain  Gain=rhoGLU
  Product : Product  RndMeth=Zero
  Sum2 : Sum  Inputs=|+-
  Sum5 : Sum  Inputs=|+-
  lmtu [m] : Outport  VectorParamsAs1DForOutWhenUnconnected=off
  lever [m] : Outport  Port=2  VectorParamsAs1DForOutWhenUnconnected=off
  wires:
  Constant/1 -> Sum5/1
  Sum5/1 -> lmtu [m]/1
  Product/1 -> Gain2/1
  phi34 [rad]/1 -> Sum2/1
  Constant2/1 -> Sum2/2
  Sum2/1 -> Product/1
  Constant1/1 -> Product/2, lever [m]/1
  Gain2/1 -> Sum5/2

== system nms_sim_2D_cost/Muscle Actuation/R HAM Link ==
  note: HAM Attachment
  phi34 [rad] : Inport
  phi23 [rad] : Inport  Port=2
  Constant1 : Constant  Value=rHAMk
  Constant2 : Constant  Value=phirefHAMk
  Constant3 : Constant  Value=rHAMh
  Constant4 : Constant  Value=lslackHAM+loptHAM
  Constant5 : Constant  Value=phirefHAMh
  Gain2 : Gain  Gain=rhoHAMh
  Gain4 : Gain  Gain=rhoHAMk
  Product : Product  RndMeth=Zero
  Product1 : Product  RndMeth=Zero
  Sum1 : Sum  Inputs=|+-
  Sum4 : Sum  Inputs=|+-
  Sum5 : Sum  Inputs=-++
  lmtu [m] : Outport  VectorParamsAs1DForOutWhenUnconnected=off
  lever34 [m] : Outport  Port=2  VectorParamsAs1DForOutWhenUnconnected=off
  lever23 [m] : Outport  Port=3  VectorParamsAs1DForOutWhenUnconnected=off
  wires:
  Sum5/1 -> lmtu [m]/1
  Constant4/1 -> Sum5/2
  Gain4/1 -> Sum5/3
  Gain2/1 -> Sum5/1
  phi34 [rad]/1 -> Sum4/1
  Constant5/1 -> Sum4/2
  Sum4/1 -> Product/1
  Constant3/1 -> Product/2, lever34 [m]/1
  Product/1 -> Gain2/1
  phi23 [rad]/1 -> Sum1/1
  Constant2/1 -> Sum1/2
  Sum1/1 -> Product1/1
  Constant1/1 -> Product1/2, lever23 [m]/1
  Product1/1 -> Gain4/1

== system nms_sim_2D_cost/Muscle Actuation/R HFL Link ==
  note: HFL Attachment
  phi34 [rad] : Inport
  Constant : Constant  Value=lslackHFL+loptHFL
  Constant1 : Constant  Value=rHFL
  Constant2 : Constant  Value=phirefHFL
  Gain2 : Gain  Gain=rhoHFL
  Product : Product  RndMeth=Zero
  Sum2 : Sum  Inputs=|+-
  Sum5 : Sum  Inputs=|++
  lmtu [m] : Outport  VectorParamsAs1DForOutWhenUnconnected=off
  lever [m] : Outport  Port=2  VectorParamsAs1DForOutWhenUnconnected=off
  wires:
  Constant/1 -> Sum5/1
  Sum5/1 -> lmtu [m]/1
  Product/1 -> Gain2/1
  phi34 [rad]/1 -> Sum2/1
  Constant2/1 -> Sum2/2
  Sum2/1 -> Product/1
  Constant1/1 -> Product/2, lever [m]/1
  Gain2/1 -> Sum5/2

== system nms_sim_2D_cost/Muscle Actuation/R Hip Joint Limits ==
  note: Hip Joint Limits
  phi [rad] : Inport
  dphi [rad/s] : Inport  Port=2
  Gain1 : Gain  Gain=c_jointstop
  Gain2 : Gain  Gain=-1
  Gain3 : Gain  Gain=c_jointstop
  Gain4 : Gain  Gain=1/w_max_jointstop
  Limit Ankle Range : simulink/Logic and Bit Operations/Interval Test  Commented=on  IntervalClosedRight=on  uplimit=phi12_UpLimit + 40*pi/180  IntervalClosedLeft=on  lowlimit=phi12_LowLimit - 40*pi/180  OutDataTypeStr=boolean
  Logical Operator3 : Logic  Commented=on  Operator=NOT  AllPortsSameDT=off  OutDataTypeStr=boolean
  Mux1 : Mux  Inputs=2
  Mux3 : Mux  Inputs=2
  Overextension Torque : Fcn  Expr="- u(1)  *  (1-u(2)) * (u(2)<1) * (u(1)>0)"
  Overflexion Torque : Fcn  Expr="- u(1)  *  (1-u(2)) * (u(2)<1) * (u(1)<0)"
  Stop Simulation1 : Stop  Commented=on
  Sum : Sum  Inputs=|+-
  Sum1 : Sum  Inputs=|+-
  Sum2 : Sum
  overextension angle : Constant  Value=phi34_UpLimit
  overflexion angle : Constant  Value=phi34_LowLimit
  M_stop [Nm] : Outport  VectorParamsAs1DForOutWhenUnconnected=off
  wires:
  Mux3/1 -> Overextension Torque/1
  Gain3/1 -> Mux3/1
  dphi [rad/s]/1 -> Gain4/1
  overextension angle/1 -> Sum/2
  phi [rad]/1 -> Sum/1, Sum1/1, Limit Ankle Range/1
  Sum/1 -> Gain3/1
  Gain4/1 -> Gain2/1, Mux1/2
  Gain1/1 -> Mux1/1
  Sum1/1 -> Gain1/1
  overflexion angle/1 -> Sum1/2
  Mux1/1 -> Overflexion Torque/1
  Sum2/1 -> M_stop [Nm]/1
  Gain2/1 -> Mux3/2
  Overflexion Torque/1 -> Sum2/2
  Overextension Torque/1 -> Sum2/1
  Limit Ankle Range/1 -> Logical Operator3/1
  Logical Operator3/1 -> Stop Simulation1/1

== system nms_sim_2D_cost/Muscle Actuation/R Knee Joint Limits ==
  note: Knee Joint Limits
  phi [rad] : Inport
  dphi [rad/s] : Inport  Port=2
  Gain1 : Gain  Gain=c_jointstop
  Gain2 : Gain  Gain=-1
  Gain3 : Gain  Gain=c_jointstop
  Gain4 : Gain  Gain=1/w_max_jointstop
  Limit Ankle Range : simulink/Logic and Bit Operations/Interval Test  Commented=on  IntervalClosedRight=on  uplimit=phi12_UpLimit + 40*pi/180  IntervalClosedLeft=on  lowlimit=phi12_LowLimit - 40*pi/180  OutDataTypeStr=boolean
  Logical Operator3 : Logic  Commented=on  Operator=NOT  AllPortsSameDT=off  OutDataTypeStr=boolean
  Mux1 : Mux  Inputs=2
  Mux3 : Mux  Inputs=2
  Overextension Torque : Fcn  Expr="- u(1)  *  (1-u(2)) * (u(2)<1) * (u(1)>0)"
  Overflexion Torque : Fcn  Expr="- u(1)  *  (1-u(2)) * (u(2)<1) * (u(1)<0)"
  Stop Simulation1 : Stop  Commented=on
  Sum : Sum  Inputs=|+-
  Sum1 : Sum  Inputs=|+-
  Sum2 : Sum
  overextension angle : Constant  Value=phi23_UpLimit
  overflexion angle : Constant  Value=phi23_LowLimit
  M_stop [Nm] : Outport  VectorParamsAs1DForOutWhenUnconnected=off
  wires:
  Mux3/1 -> Overextension Torque/1
  Gain3/1 -> Mux3/1
  dphi [rad/s]/1 -> Gain4/1
  overextension angle/1 -> Sum/2
  phi [rad]/1 -> Sum/1, Sum1/1, Limit Ankle Range/1
  Sum/1 -> Gain3/1
  Gain4/1 -> Gain2/1, Mux1/2
  Gain1/1 -> Mux1/1
  Sum1/1 -> Gain1/1
  overflexion angle/1 -> Sum1/2
  Mux1/1 -> Overflexion Torque/1
  Sum2/1 -> M_stop [Nm]/1
  Gain2/1 -> Mux3/2
  Overflexion Torque/1 -> Sum2/2
  Overextension Torque/1 -> Sum2/1
  Limit Ankle Range/1 -> Logical Operator3/1
  Logical Operator3/1 -> Stop Simulation1/1
